simulink model "closeloop_fyp_finalllllll_2025a"  (R2025b)
settings: Solver=FixedStepAuto  StartTime=0.0  StopTime=15  FixedStep=5e-6  RelTol=1e-3
undefined symbols (not defined in the file): Ion, Lithium
libraries: spsMosfetLib x16, spsSeriesRLCBranchLib x12, spsCurrentMeasurementLib x5, spsVoltageMeasurementLib x5, spsBatteryLib x2, spsLinearTransformerLib x1, dspstat3 x1, slpidlib x1, simulink x1, spsTriangleGeneratorLib x1, sps_lib x1
settings Model: Creator=tanuj  LastModifiedBy=lenovo
settings SolverCC: ZeroCrossControl=DisableAll  ZeroCrossAlgorithm=Adaptive
settings DataIOCC: SaveOperatingPoint=on  Refine=2
settings DebuggingCC: MaskedZcDiagnostic=none  IgnoredZcDiagnostic=none

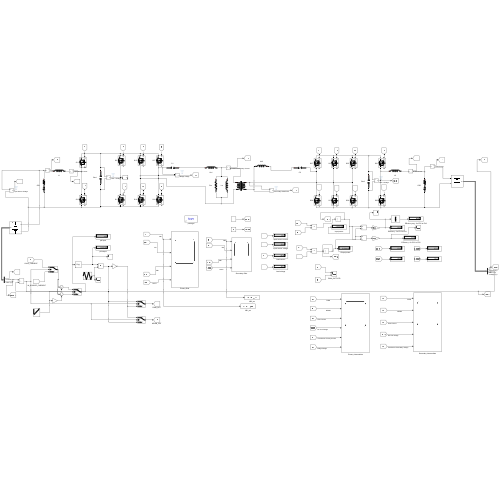
[thumbnail: Simulink's stored preview of the top-level diagram]
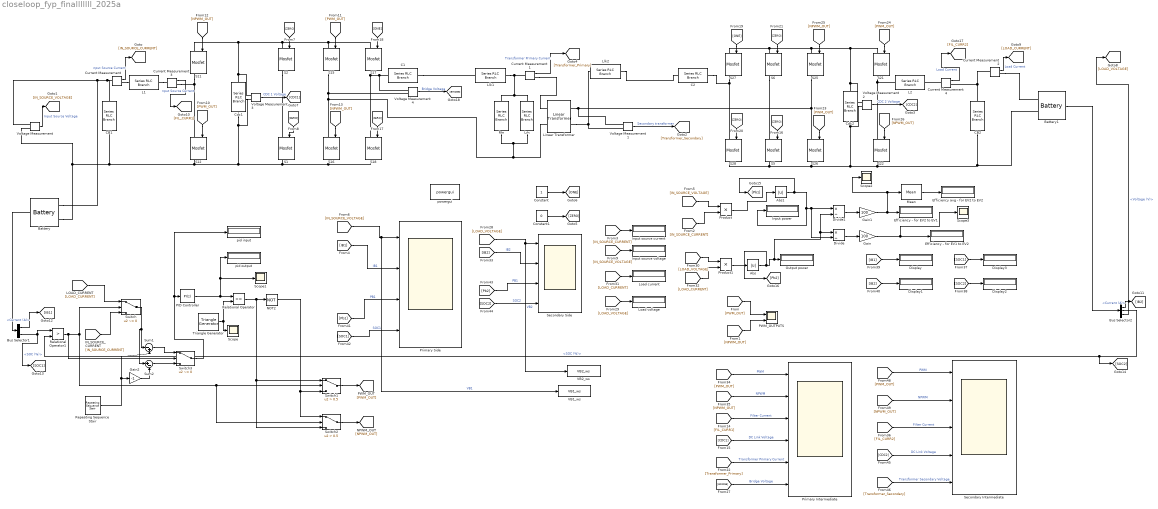
== system closeloop_fyp_finalllllll_2025a ==
  Abs : Abs  SaturateOnIntegerOverflow=off
  Abs1 : Abs  SaturateOnIntegerOverflow=off
  Battery : spsBatteryLib/Battery  BatType=Lithium-Ion  NomV=350  NomQ=60  SOC=25  Batt_Tr=30  PresetModel=on  MaxQ=60  MinV=262.5  FullV=407.3955  Dis_rate=26.087  R=0.058333  Normal_OP=54.2609  expZone="[378.135      2.947826]"
  Battery1 : spsBatteryLib/Battery  BatType=Lithium-Ion  NomV=450  NomQ=80  SOC=75  Batt_Tr=30  PresetModel=off  MaxQ=80  MinV=337.5  FullV=523.7942  Dis_rate=34.7826  R=0.05625  Normal_OP=72.3478  expZone="[486.1736      3.930435]"
  Bus Selector1 : BusSelector  OutputSignals=Current (A),SOC (%)
  Bus Selector2 : BusSelector  OutputSignals=Current (A),SOC (%),Voltage (V)
  "C1 " : spsSeriesRLCBranchLib/Series RLC Branch  LConnTagsString=__new0  RConnTagsString=__new0  BranchType=C  Resistance=1  Inductance=1e-3  SetiL0=off  InitialCurrent=0  Capacitance=0.21e-3  Setx0=off  InitialVoltage=0  Measurements=None
  C2 : spsSeriesRLCBranchLib/Series RLC Branch  LConnTagsString=__new0  RConnTagsString=__new0  BranchType=C  Resistance=1  Inductance=1e-3  SetiL0=off  InitialCurrent=0  Capacitance=0.21e-3  Setx0=off  InitialVoltage=0  Measurements=None
  CB1 : spsSeriesRLCBranchLib/Series RLC Branch  LConnTagsString=__new0  RConnTagsString=__new0  BranchType=RC  Resistance=0.01  Inductance=1e-3  SetiL0=off  InitialCurrent=0  Capacitance=1.6e-6  Setx0=off  InitialVoltage=350  Measurements=None
  CB2 : spsSeriesRLCBranchLib/Series RLC Branch  LConnTagsString=__new0  RConnTagsString=__new0  BranchType=RC  Resistance=0.01  Inductance=1e-3  SetiL0=off  InitialCurrent=0  Capacitance=1.8e-6  Setx0=off  InitialVoltage=0  Measurements=None
  Cdc1 : spsSeriesRLCBranchLib/Series RLC Branch  LConnTagsString=__new0  RConnTagsString=__new0  BranchType=C  Resistance=1  Inductance=1e-3  SetiL0=off  InitialCurrent=0  Capacitance=0.5e-3  Setx0=off  InitialVoltage=350  Measurements=None
  Cdc2 : spsSeriesRLCBranchLib/Series RLC Branch  LConnTagsString=__new0  RConnTagsString=__new0  BranchType=C  Resistance=1  Inductance=1e-3  SetiL0=off  InitialCurrent=0  Capacitance=0.8e-3  Setx0=off  InitialVoltage=450  Measurements=None
  Constant : Constant
  Constant1 : Constant  Value=0
  Current Measurement{,1..4} (5 alike) : spsCurrentMeasurementLib/Current Measurement  PhasorSimulation=off  OutputType=Complex  PSBequivalent=0
  Display{,1..3} (4 alike) : Display
  Divide : Product  Inputs=*/
  Divide1 : Product  Inputs=*/
  Efficiency - for EV1 to EV2 : Display
  Efficiency - for EV2 to EV1 : Display
  Efficiency avg - for EV2 to EV2 : Display
  Gain : Gain  Gain=100
  Gain1 : Gain  Gain=100
  Gain2 : Gain  Gain=-1
  Input power : Display
  Input source current : Display
  Input source voltage : Display
  L1 : spsSeriesRLCBranchLib/Series RLC Branch  LConnTagsString=__new0  RConnTagsString=__new0  BranchType=L  Resistance=1  Inductance=1.11e-3  SetiL0=off  InitialCurrent=0  Capacitance=1e-6  Setx0=off  InitialVoltage=0  Measurements=None
  L2 : spsSeriesRLCBranchLib/Series RLC Branch  LConnTagsString=__new0  RConnTagsString=__new0  BranchType=L  Resistance=1  Inductance=1.15e-3  SetiL0=off  InitialCurrent=40  Capacitance=1e-6  Setx0=off  InitialVoltage=0  Measurements=None
  Linear Transformer : spsLinearTransformerLib/Linear Transformer  UNITS=pu  NominalPower=[24000 50000]  winding1=[350 0.02 0.01]  winding2=[450 0.002 0.01]  ThreeWindings=off  winding3=[ 315e3 0.002 0.08 ]  RmLm=[500 500]  Measurements=None  DataType=off
  Llk1 : spsSeriesRLCBranchLib/Series RLC Branch  LConnTagsString=__new0  RConnTagsString=__new0  BranchType=L  Resistance=1  Inductance=0.3015e-6  SetiL0=off  InitialCurrent=0  Capacitance=1e-6  Setx0=off  InitialVoltage=0  Measurements=None
  Llk2 : spsSeriesRLCBranchLib/Series RLC Branch  LConnTagsString=__new0  RConnTagsString=__new0  BranchType=L  Resistance=1  Inductance=0.3015e-6  SetiL0=off  InitialCurrent=0  Capacitance=1e-6  Setx0=off  InitialVoltage=0  Measurements=None
  Lm : spsSeriesRLCBranchLib/Series RLC Branch  LConnTagsString=__new0  RConnTagsString=__new0  BranchType=L  Resistance=1  Inductance=2.2725e-3  SetiL0=off  InitialCurrent=0  Capacitance=1e-6  Setx0=off  InitialVoltage=0  Measurements=None
  Load current : Display
  Load voltage : Display
  Mean : dspstat3/Mean  run=off  InputProcessing=Columns as channels (frame based)  reset_popup=None  directionMode=Each column  dimension=1  roiEnable=off  roiType=Rectangles  roiPortion=Entire ROI  roiOutput=Individual statistics for each ROI  roiFlag=off  roundingMode=Floor  overflowMode=off  outputDataTypeStr=Inherit: Same as accumulator  outputMin=[]  outputMax=[]  outputLastDataTypeStr=Inherit: Same as accumulator
  NOT2 : Logic  Operator=NOT  IconShape=distinctive  AllPortsSameDT=off  OutDataTypeStr=boolean
  Output power : Display
  PID Controller : slpidlib/PID Controller  Controller=PI  Form=Parallel  TimeDomain=Discrete-time  UseExternalTs=off  SampleTime=-1  IntegratorMethod=Forward Euler  FilterMethod=Forward Euler  ControllerParametersSource=internal  P=0.0001  I=0.015  UseKiTs=off  D=0  UseExternalDerivativeSource=off  N=100  UseFilter=on  TunerSelectOption=Transfer Function Based (PID Tuner App)  InitialConditionSource=internal  InitialConditionForIntegrator=0  InitialConditionForFilter=0  DifferentiatorICPrevScaledInput=0  ExternalReset=none  TrackingMode=off  Kt=1  LimitOutput=off  SatLimitsSource=internal  UpperSaturationLimit=0.95  LowerSaturationLimit=0.01  LinearizeAsGain=on  AntiWindupMode=none  Kb=1  LimitIntegrator=off  UpperIntegratorSaturationLimit=inf  LowerIntegratorSaturationLimit=-inf  POutMin=[]  POutMax=[]  IOutMin=[]  IOutMax=[]  DOutMin=[]  DOutMax=[]  NOutMin=[]  NOutMax=[]  SumOutMin=[]  SumOutMax=[]  SaturationOutMin=[]  SaturationOutMax=[]  PParamMin=[]  PParamMax=[]  IParamMin=[]  IParamMax=[]  DParamMin=[]  DParamMax=[]  NParamMin=[]  NParamMax=[]  KbParamMin=[]  KbParamMax=[]  KtParamMin=[]  KtParamMax=[]  KbOutMin=[]  KbOutMax=[]  KtOutMin=[]  KtOutMax=[]  IntegratorOutMin=[]  IntegratorOutMax=[]  FilterOutMin=[]  FilterOutMax=[]  SumI1OutMin=[]  SumI1OutMax=[]  SumI2OutMin=[]  SumI2OutMax=[]  SumI3OutMin=[]  SumI3OutMax=[]  SumI4OutMin=[]  SumI4OutMax=[]  SumDOutMin=[]  SumDOutMax=[]  DifferentiatorOutMin=[]  DifferentiatorOutMax=[]  FilterDiffOutCoefMin=[]  FilterDiffOutCoefMax=[]  ReciprocalOutMin=[]  ReciprocalOutMax=[]  SumDenOutMin=[]  SumDenOutMax=[]  SumNumOutMin=[]  SumNumOutMax=[]  DivideOutMin=[]  DivideOutMax=[]  UdiffTsProdOutMin=[]  UdiffTsProdOutMax=[]  NTsProdOutMin=[]  NTsProdOutMax=[]  UintegralTsProdOutMin=[]  UintegralTsProdOutMax=[]  UngainTsProdOutMin=[]  UngainTsProdOutMax=[]  ClampingZeroOutDataTypeStr=Inherit: Inherit via back propagation  ClampingZeroOutMin=[]  ClampingZeroOutMax=[]  FilterDenConstantOutDataTypeStr=Inherit: Inherit via back propagation  FilterDenConstantOutMin=[]  FilterDenConstantOutMax=[]  PCopyOutDataTypeStr=Inherit: Inherit via back propagation  PCopyOutMin=[]  PCopyOutMax=[]  NCopyOutDataTypeStr=Inherit: Inherit via back propagation  NCopyOutMin=[]  NCopyOutMax=[]  IntegratorContinuousStateAttributes=''  IntegratorStateMustResolveToSignalObject=off  IntegratorRTWStateStorageClass=Auto  FilterContinuousStateAttributes=''  FilterStateMustResolveToSignalObject=off  FilterRTWStateStorageClass=Auto  ParallelPVariant=InternalParameters  IdealPVariant=Disabled  IVariant=InternalParameters  DVariant=Disabled  IntegratorVariant=Discrete  SatVariant=Disabled  AWVariant=Passthrough  PCopyVariant=Disabled  TRVariant=Disabled  FdbkBlocksVariant=Forward  IdealPFdbkVariant=Disabled  SatFdbkVariant=Disabled  DerivativeFilterVariant=Disabled  NVariant=Disabled  NCopyVariant=Disabled_SignalSpec  FilterICVariant=Disabled  IntegratorICVariant=InternalICs  ExternalResetVariant=Disabled  TRSumVariant=Passthrough  SumFdbkVariant=Disabled  SumVariant=Sum_PI  TsampFilterVariant=InternalTs  TsampNgainVariant=Passthrough  TsampIntegralVariant=Disabled_SignalSpec  ExternalSaturationOutDataTypeStr=Inherit: Same as second input  DerivativeSourceVariant=Disabled  PreIntVariant=InternalPreInt
  PWM_OUTPUTS : Scope  NumInputPorts=2
      settings: ActiveDisplayYMinimum=-0.125  ActiveDisplayYMaximum=1.125  DataLoggingVariableName=ScopeData3
  Primary Intermediate : Scope  NumInputPorts=6
      settings: ActiveDisplayString=6  ActiveDisplayYMinimum=-98.1980175081683  ActiveDisplayYMaximum=834.82790101932073  DataLoggingVariableName=ScopeData7
  Primary Side : Scope  NumInputPorts=4
      settings: ActiveDisplayYMinimum=372.10737831413792  ActiveDisplayYMaximum=377.5563352303227
  Product : Product
  Product1 : Product
  Relational Operator : RelationalOperator  OutDataTypeStr=boolean  RndMeth=Simplest  InputSameDT=off
  Relational Operator1 : RelationalOperator  Operator=>  OutDataTypeStr=boolean  RndMeth=Simplest  InputSameDT=off
  Repeating Sequence Stair : simulink/Sources/Repeating Sequence Stair  OutValues=[10 20 30 40 50].'  tsamp=3  OutMin=[]  OutMax=[]  OutDataTypeStr=double  OutputDataTypeScalingMode=double  OutDataType=fixdt(0,8)  ConRadixGroup=Best Precision: Vector-wise  OutScaling=2^-12
  Rm : spsSeriesRLCBranchLib/Series RLC Branch  LConnTagsString=__new0  RConnTagsString=__new0  BranchType=R  Resistance=500  Inductance=1e-3  SetiL0=off  InitialCurrent=0  Capacitance=1e-6  Setx0=off  InitialVoltage=0  Measurements=None
  S{1..2,5..6,11..12,15..17,21..22,25..28} (15 alike) : spsMosfetLib/Mosfet  Ron=0.1  Lon=0  Rd=0.01  Vfd=0  IC=0  Rs=1e5  Cs=inf  Measurements=on
  S18 : spsMosfetLib/Mosfet  Ron=0.2  Lon=0  Rd=0.2  Vfd=0  IC=0  Rs=1e5  Cs=inf  Measurements=on
  Scope{,1..3} (4 alike) : Scope
      Scope settings: ActiveDisplayYMinimum=-0.125  ActiveDisplayYMaximum=1.125  DataLoggingVariableName=ScopeData2
      Scope1 settings: ActiveDisplayYMinimum=-0.0011237  ActiveDisplayYMaximum=0.00049866  DataLoggingVariableName=ScopeData4
      Scope2 settings: ActiveDisplayYMinimum=-2.7085044653E+6  ActiveDisplayYMaximum=2.43765402009E+7  DataLoggingVariableName=ScopeData5
      Scope3 settings: DataLoggingVariableName=ScopeData6
  Secondary Intermediate : Scope  NumInputPorts=5
      settings: ActiveDisplayString=5  ActiveDisplayYMinimum=-608.33508488052962  ActiveDisplayYMaximum=602.59865992099026  DataLoggingVariableName=ScopeData8
  Secondary Side : Scope  NumInputPorts=4
      settings: ActiveDisplayYMinimum=482.29640761876993  ActiveDisplayYMaximum=487.73451877626997
  Sum1 : Sum  Inputs=|-+
  Sum2 : Sum  Inputs=|+-
  Switch : Switch  Criteria=u2 ~= 0  Threshold=0.5  SaturateOnIntegerOverflow=off  InputSameDT=off
  Switch1 : Switch  Criteria=u2 > Threshold  Threshold=0.5  SaturateOnIntegerOverflow=off  InputSameDT=off
  Switch2 : Switch  Criteria=u2 > Threshold  Threshold=0.5  SaturateOnIntegerOverflow=off  InputSameDT=off
  Switch3 : Switch  Criteria=u2 ~= 0  Threshold=0.5  SaturateOnIntegerOverflow=off  InputSameDT=off
  Triangle Generator : spsTriangleGeneratorLib/Triangle Generator  Freq=25000  Phase=90  Ts=0
  VB1_ws : ToWorkspace  VariableName=VB1_ws  SaveFormat=Timeseries  SampleTime=-1
  VB2_ws : ToWorkspace  VariableName=VB2_ws  SaveFormat=Timeseries  SampleTime=-1
  Voltage Measurement{,1..4} (5 alike) : spsVoltageMeasurementLib/Voltage Measurement  PhasorSimulation=off  OutputType=Complex  PSBequivalent=0
  pid input : Display
  pid output : Display
  powergui : sps_lib/powergui  Priority=1  SimulationMode=Discrete  SampleTime=5e-6  frequency=60  Iterations=50  frequencyindice=0  Pbase=100e6  ErrMax=1e-4  UnitsV=kV  UnitsW=MW  buscounter=0  FunctionMessages=off  echomessages=off  EnableUseOfTLC=off  CurrentSourceSwitches=off  DisableSnubberDevices=off  DisableRonSwitches=off  DisableVfSwitches=off  DisplayEquations=off  AutomaticDiscreteSolvers=off  SolverType=Tustin/Backward Euler (TBE)  Interpol=off  ExternalGateDelay=off  methode=off  Ts=100  x0status=blocks  SPID=on  SwTol=0  HookPort=off  NonlinearTolerance=1e-4  nMaxIteration=100  ContinueOnMaxIteration=off  RestoreLinks=warning  ResistiveCurrentMeasurement=off  Frange=[0:2:500]  Ylog=off  Xlog=on  ShowGrid=off  save=off  variable=ZData  structure=0  ZoomFFT=off  StartTime=0.0  cycles=1  DisplayStyle=1  fundamental=60  FreqAxis=off  MaxFrequency=1000  frequencyindicesteady=1  RmsSteady=1  display=off
  wires:
  Product/1 -> Abs1/1
  Product1/1 -> Abs/1
  Battery/1 -> Bus Selector1/1
  Battery1/1 -> Bus Selector2/1
  Switch/1 -> Sum2/1, Sum1/1
  Triangle Generator/1 -> Relational Operator/2, Scope/1
  Relational Operator/1 -> Switch2/3, Switch1/1, NOT2/1
  Switch1/1 -> [PWM_OUT]
  Switch2/1 -> [NPWM_OUT]
  [PWM_OUT] -> PWM_OUTPUTS/1
  [NPWM_OUT] -> PWM_OUTPUTS/2
  Current Measurement/1 -> [IN_SOURCE_CURRENT]  "nput Source Current"
  [IN_SOURCE_CURRENT] -> Product/2
  [IN_SOURCE_CURRENT] -> Input source current/1
  [IB1] -> Primary Side/2  "IB1"
  Voltage Measurement/1 -> [IN_SOURCE_VOLTAGE]  "Input Source Voltage"
  [IN_SOURCE_VOLTAGE] -> Product/1
  [IN_SOURCE_VOLTAGE] -> VB1_ws/1, Primary Side/1  "VB1"
  [IN_SOURCE_VOLTAGE] -> Input source voltage/1
  [PWM_OUT] -> S12/1
  [PWM_OUT] -> S15/1
  [NPWM_OUT] -> S11/1
  [NPWM_OUT] -> S16/1
  Constant1/1 -> [ZERO]
  [ZERO] -> S18/1
  Constant/1 -> [ONE]
  [ONE] -> S17/1
  [ONE] -> S27/1
  [ZERO] -> S28/1
  [PWM_OUT] -> S26/1
  [PWM_OUT] -> S21/1
  [NPWM_OUT] -> S22/1
  [NPWM_OUT] -> S25/1
  Current Measurement2/1 -> [LOAD_CURRENT]  "Load Current"
  [LOAD_VOLTAGE] -> Load voltage/1
  [LOAD_VOLTAGE] -> Product1/1
  [LOAD_CURRENT] -> Load current/1
  [LOAD_CURRENT] -> Product1/2
  [IB2] -> Secondary Side/2  "IB2"
  [LOAD_VOLTAGE] -> VB2_ws/1, Secondary Side/1  "VB2"
  Divide/1 -> Gain/1
  Bus Selector1/2 -> Relational Operator1/1, [SOC1]  "<SOC (%)>"
  Bus Selector2/2 -> Relational Operator1/2, [SOC2]  "<SOC (%)>"
  Bus Selector2/1 -> [IB2]  "<Current (A)>"
  Bus Selector1/1 -> [IB1]  "<Current (A)>"
  [IN_SOURCE_CURRENT] -> Switch/3
  [SOC1] -> Display3/1
  [SOC2] -> Display2/1
  [IB1] -> Display/1
  [IB2] -> Display1/1
  Relational Operator1/1 -> Switch2/2, Switch1/2, Switch/2, Switch3/2
  Bus Selector2/3 -> [LOAD_VOLTAGE]  "<Voltage (V)>"
  PID Controller/1 -> pid output/1, Scope1/1, Relational Operator/1
  [Pb1] -> Primary Side/3  "PB1"
  [SOC1] -> Primary Side/4  "SOC1"
  [Pb2] -> Secondary Side/3  "PB1"
  [SOC2] -> Secondary Side/4  "SOC2"
  NOT2/1 -> Switch2/1, Switch1/3
  Divide1/1 -> Gain1/1
  Gain1/1 -> Mean/1, Scope2/1, Efficiency - for EV2 to EV1/1
  Abs/1 -> [Pb2], Divide/1, Divide1/2, Output power/1
  Abs1/1 -> Divide/2, Divide1/1, Input power/1, [Pb1]
  Gain/1 -> Scope3/1, Efficiency - for EV1 to EV2/1
  Mean/1 -> Efficiency avg - for EV2 to EV2/1
  [LOAD_CURRENT] -> Switch/1
  Repeating Sequence Stair/1 -> Gain2/1, Sum1/2
  Sum1/1 -> Switch3/1
  Sum2/1 -> Switch3/3
  Gain2/1 -> Sum2/2
  Switch3/1 -> pid input/1, PID Controller/1
  [ZERO] -> S2/1
  [ZERO] -> S1/1
  [ZERO] -> S5/1
  [ZERO] -> S6/1
  Voltage Measurement1/1 -> [Transformer_Secondary]  "Secondary transformer"
  Voltage Measurement2/1 -> [CDC2]  "CDC 2 Voltage"
  Current Measurement1/1 -> [Transformer_Primary]  "Transformer Primary Current"
  Voltage Measurement3/1 -> [CDC1]  "CDC 1 Voltage"
  Current Measurement3/1 -> [FIL_CURR1]  "nput Source Current"
  Current Measurement4/1 -> [FIL_CURR2]  "Load Current"
  Voltage Measurement4/1 -> [BRIDGE]  "Bridge Voltage"
  [FIL_CURR1] -> Primary Intermediate/3  "Filter Current"
  [CDC1] -> Primary Intermediate/4  "DC Link Voltage"
  [Transformer_Primary] -> Primary Intermediate/5  "Transformer Primary Current"
  [BRIDGE] -> Primary Intermediate/6  "Bridge Voltage"
  [PWM_OUT] -> Primary Intermediate/1  "PWM"
  [NPWM_OUT] -> Primary Intermediate/2  "NPWM"
  [Transformer_Secondary] -> Secondary Intermediate/5  "Transformer Secondary Voltage"
  [CDC2] -> Secondary Intermediate/4  "DC Link Voltage"
  [NPWM_OUT] -> Secondary Intermediate/2  "NPWM"
  [FIL_CURR2] -> Secondary Intermediate/3  "Filter Current"
  [PWM_OUT] -> Secondary Intermediate/1  "PWM"
  connections:
  S12/RConn1 -- Voltage Measurement3/LConn2 -- Cdc1/RConn1 -- S1/RConn1 -- S18/RConn1 -- S16/RConn1 -- Voltage Measurement/LConn2 -- Battery/LConn2 -- CB1/RConn1
  L1/RConn1 -- Current Measurement3/LConn1
  S15/RConn1 -- S16/LConn1 -- Linear Transformer/LConn2 -- Lm/RConn1 -- Rm/RConn1 -- Voltage Measurement4/LConn2
  S17/RConn1 -- Voltage Measurement4/LConn1 -- "C1 "/RConn1 -- S18/LConn1
  "C1 "/LConn1 -- Llk1/LConn1
  Rm/LConn1 -- Llk1/RConn1 -- Current Measurement1/LConn1 -- Lm/LConn1
  Llk2/LConn1 -- C2/LConn1
  Linear Transformer/RConn2 -- Llk2/RConn1 -- Voltage Measurement1/LConn2
  S27/RConn1 -- S28/LConn1 -- C2/RConn1
  S25/RConn1 -- Voltage Measurement1/LConn1 -- Linear Transformer/RConn1 -- S26/LConn1
  S21/RConn1 -- S22/LConn1 -- L2/LConn1
  S27/LConn1 -- S6/LConn1 -- S25/LConn1 -- Cdc2/LConn1 -- Voltage Measurement2/LConn1 -- S21/LConn1
  S28/RConn1 -- S5/RConn1 -- S26/RConn1 -- Voltage Measurement2/LConn2 -- Cdc2/RConn1 -- Battery1/LConn2 -- CB2/RConn1 -- S22/RConn1
  CB2/LConn1 -- Current Measurement2/LConn1 -- Current Measurement4/RConn1
  Current Measurement/RConn1 -- L1/LConn1
  Current Measurement1/RConn1 -- Linear Transformer/LConn1
  CB1/LConn1 -- Battery/LConn1 -- Voltage Measurement/LConn1 -- Current Measurement/LConn1
  Current Measurement2/RConn1 -- Battery1/LConn1
  S17/LConn1 -- S15/LConn1 -- S2/LConn1 -- S11/LConn1 -- Voltage Measurement3/LConn1 -- Cdc1/LConn1
  S2/RConn1 -- S1/LConn1
  S6/RConn1 -- S5/LConn1
  Current Measurement3/RConn1 -- S11/RConn1 -- S12/LConn1
  Current Measurement4/LConn1 -- L2/RConn1
